simulink model "cable_driven_parallel_robot2022"  (R2022b)
settings: Solver=ode3  StartTime=0.0  StopTime=100  FixedStep=0.01  RelTol=1e-3
values from neighbouring files (symbols this model uses):
  cable_length = 1.2    [Model_Info.m]
  g = 9.81    [Model_Info.m]
  MP_H = 2    [Model_Info.m]
  MP_init_X = 0    [Model_Info.m]
  MP_init_Y = 0    [Model_Info.m]
  MP_init_Z = cable_length + (MP_H/2)    (= 2.2)    [Model_Info.m]
  MP_Ix = (MP_m/12)*(MP_W^2+MP_H^2)    (= 6.66666666667e-05)    [Model_Info.m]
  MP_Iy = (MP_m/12)*(MP_L^2+MP_H^2)    (= 6.66666666667e-05)    [Model_Info.m]
  MP_Iz = (MP_m/12)*(MP_L^2+MP_W^2)    (= 6.66666666667e-05)    [Model_Info.m]
  MP_L = 2    [Model_Info.m]
  MP_m = 0.0001    [Model_Info.m]
  MP_W = 2    [Model_Info.m]
  MR_init_X_L1 = -(MP_L/2)    (= -1)    [Model_Info.m]
  MR_init_X_L2 = (MP_L/2)    (= 1)    [Model_Info.m]
  MR_init_X_L3 = (MP_L/2)    (= 1)    [Model_Info.m]
  MR_init_X_L4 = -(MP_L/2)    (= -1)    [Model_Info.m]
  MR_init_Y_L1 = -(MP_W/2)    (= -1)    [Model_Info.m]
  MR_init_Y_L2 = -(MP_W/2)    (= -1)    [Model_Info.m]
  MR_init_Y_L3 = (MP_W/2)    (= 1)    [Model_Info.m]
  MR_init_Y_L4 = (MP_W/2)    (= 1)    [Model_Info.m]
  MR_init_Yaw_L1 = pi    (= 3.14159265359)    [Model_Info.m]
  MR_init_Yaw_L2 = 0    [Model_Info.m]
  MR_init_Yaw_L3 = 0    [Model_Info.m]
  MR_init_Yaw_L4 = pi    (= 3.14159265359)    [Model_Info.m]
  MR_Jr = (MR_m/12)*(MR_L^2+MR_W^2)    (= 0.333333333333)    [Model_Info.m]
  MR_m = 0.5    [Model_Info.m]
  MR_r = 2    [Model_Info.m]
  MR_WT = 2    [Model_Info.m]
  QR_Ax = 0.25*0    (= 0)    [Model_Info.m]
  QR_Ay = 0.25*0    (= 0)    [Model_Info.m]
  QR_Az = 0.25*0    (= 0)    [Model_Info.m]
  QR_b = 1.14*1e-7    (= 1.14e-07)    [Model_Info.m]
  QR_Ixx = 4.856*1e-3    (= 0.004856)    [Model_Info.m]
  QR_Iyy = 4.856*1e-3    (= 0.004856)    [Model_Info.m]
  QR_Izz = 8.801*1e-3    (= 0.008801)    [Model_Info.m]
  QR_K = 2.980*1e-6    (= 2.98e-06)    [Model_Info.m]
  QR_l = 0.225    [Model_Info.m]
  QR_m = 0.468    [Model_Info.m]
  QR_x0_U1 = -(MP_L/2)    (= -1)    [Model_Info.m]
  QR_x0_U2 = (MP_L/2)    (= 1)    [Model_Info.m]
  QR_x0_U3 = (MP_L/2)    (= 1)    [Model_Info.m]
  QR_x0_U4 = -(MP_L/2)    (= -1)    [Model_Info.m]
  QR_y0_U1 = -(MP_W/2)    (= -1)    [Model_Info.m]
  QR_y0_U2 = -(MP_W/2)    (= -1)    [Model_Info.m]
  QR_y0_U3 = (MP_W/2)    (= 1)    [Model_Info.m]
  QR_y0_U4 = (MP_W/2)    (= 1)    [Model_Info.m]
  QR_z0_U1 = 2*cable_length+(MP_H)    (= 4.4)    [Model_Info.m]
  QR_z0_U2 = 2*cable_length+(MP_H)    (= 4.4)    [Model_Info.m]
  QR_z0_U3 = 2*cable_length+(MP_H)    (= 4.4)    [Model_Info.m]
  QR_z0_U4 = 2*cable_length+(MP_H)    (= 4.4)    [Model_Info.m]
(part 8 of 12)

== matlab function cable_driven_parallel_robot2022/Actuators-CableTension-MovingPlatform/QuadRotor3/Subsystem/QuadCopter Model ==
  data: vx input; x_ddot output size=1; vy input; vz input; phidot input; thetadot input; psidot input; y_ddot output size=1; z_ddot output size=1; phi_ddot output size=1; theta_ddot output size=1; psi_ddot output size=1; phi input; theta input; psi input; constants input; z input; rest output
function [x_ddot,y_ddot,z_ddot,phi_ddot,theta_ddot,psi_ddot,rest] = fcn(vx,vy,vz,phidot,thetadot,psidot, phi,theta,psi,constants,z)
rest=0;
m = constants(1);
g = constants(2);
Ixx = constants(3);
Iyy = constants(4);
Izz = constants(5);
l = constants(6);
K = constants(7);
b = constants(8);
Ax = constants(9);
Ay = constants(10);
Az = constants(11);
omega1 = constants(12);
omega2 = constants(13);
omega3 = constants(14);
omega4 = constants(15);
Tx = constants(16);
Ty = constants(17);
Tz = constants(18);
% x_ddot = (K*omega1^2*sin(phi)*sin(psi) - Ax*vx + K*omega2^2*sin(phi)*sin(psi) + K*omega3^2*sin(phi)*sin(psi) + K*omega4^2*sin(phi)*sin(psi) + K*omega1^2*cos(phi)*cos(psi)*sin(theta) + K*omega2^2*cos(phi)*cos(psi)*sin(theta) + K*omega3^2*cos(phi)*cos(psi)*sin(theta) + K*omega4^2*cos(phi)*cos(psi)*sin(theta))/m;
% y_ddot = -(Ay*vy + K*omega1^2*cos(psi)*sin(phi) + K*omega2^2*cos(psi)*sin(phi) + K*omega3^2*cos(psi)*sin(phi) + K*omega4^2*cos(psi)*sin(phi) - K*omega1^2*cos(phi)*sin(psi)*sin(theta) - K*omega2^2*cos(phi)*sin(psi)*sin(theta) - K*omega3^2*cos(phi)*sin(psi)*sin(theta) - K*omega4^2*cos(phi)*sin(psi)*sin(theta))/m;
% z_ddot = (K*cos(phi)*cos(theta)*omega1^2 + K*cos(phi)*cos(theta)*omega2^2 + K*cos(phi)*cos(theta)*omega3^2 + K*cos(phi)*cos(theta)*omega4^2 - Az*vz - g*m)/m;
% phi_ddot = (2*Ixx*Iyy*b*omega1^2*sin(theta) - 2*Ixx*Iyy*b*omega2^2*sin(theta) + 2*Ixx*Iyy*b*omega3^2*sin(theta) - 2*Ixx*Iyy*b*omega4^2*sin(theta) + 2*Iyy^3*psidot^2*cos(phi)*cos(theta)^4*sin(phi)^3 - 2*Iyy^3*psidot^2*cos(phi)*cos(theta)^4*sin(phi)^5 - 2*Iyy^3*psidot*thetadot*cos(theta)^3*sin(phi)^2 + 2*Iyy^3*psidot*thetadot*cos(theta)^3*sin(phi)^4 - 2*Iyy^3*psidot^2*cos(phi)^3*cos(theta)^4*sin(phi)^3 - Iyy^3*thetadot^2*sin(2*phi)*cos(theta)^2*sin(phi)^2 + Iyy^3*thetadot^2*sin(2*phi)*cos(theta)^2*sin(phi)^4 - Ixx*Iyy^2*thetadot^2*sin(2*phi)*sin(theta)^2 - 2*Iyy^2*K*l*omega2^2*cos(theta)^2*sin(phi)^2 + 2*Iyy^2*K*l*omega2^2*cos(theta)^2*sin(phi)^4 + 2*Iyy^2*K*l*omega4^2*cos(theta)^2*sin(phi)^2 - 2*Iyy^2*K*l*omega4^2*cos(theta)^2*sin(phi)^4 + 2*Ixx*Iyy^2*thetadot^2*cos(phi)*sin(phi)*sin(theta)^2 - 2*Ixx*Iyy*b*omega1^2*sin(phi)^2*sin(theta) + 2*Ixx*Iyy*b*omega2^2*sin(phi)^2*sin(theta) - 2*Ixx*Iyy*b*omega3^2*sin(phi)^2*sin(theta) + 2*Ixx*Iyy*b*omega4^2*sin(phi)^2*sin(theta) + 2*Ixx*Izz*b*omega1^2*sin(phi)^2*sin(theta) - 2*Ixx*Izz*b*omega2^2*sin(phi)^2*sin(theta) + 2*Ixx*Izz*b*omega3^2*sin(phi)^2*sin(theta) - 2*Ixx*Izz*b*omega4^2*sin(phi)^2*sin(theta) - 2*Ixx*Iyy^2*psidot*thetadot*cos(theta)*sin(theta)^2 + 2*Ixx^2*Iyy*psidot*thetadot*cos(theta)*sin(theta)^2 + 2*Ixx*Iyy^2*psidot*thetadot*sin(2*theta)*sin(theta) - 2*Ixx^2*Iyy*psidot*thetadot*sin(2*theta)*sin(theta) - 2*Iyy*Izz^2*psidot^2*cos(phi)^3*cos(theta)^4*sin(phi) - 2*Iyy^2*Izz*psidot^2*cos(phi)*cos(theta)^4*sin(phi)^3 + 2*Iyy^2*Izz*psidot^2*cos(phi)^3*cos(theta)^4*sin(phi) - 2*Iyy*Izz^2*psidot^2*cos(phi)*cos(theta)^4*sin(phi)^5 + 4*Iyy^2*Izz*psidot^2*cos(phi)*cos(theta)^4*sin(phi)^5 - 2*Ixx*Iyy^2*thetadot^2*cos(phi)*sin(phi)^3*sin(theta)^2 - 2*Ixx*Izz^2*thetadot^2*cos(phi)*sin(phi)^3*sin(theta)^2 + Ixx*Iyy*Izz*thetadot^2*sin(2*phi)*sin(theta)^2 + 6*Iyy^3*psidot*thetadot*cos(phi)^2*cos(theta)^3*sin(phi)^2 - 4*Iyy^3*psidot*thetadot*cos(phi)^2*cos(theta)^3*sin(phi)^4 - 4*Iyy^3*psidot*thetadot*cos(phi)^4*cos(theta)^3*sin(phi)^2 + 2*Iyy*Izz^2*psidot*thetadot*cos(phi)^2*cos(theta)^3 - 2*Iyy^2*Izz*psidot*thetadot*cos(phi)^2*cos(theta)^3 - 4*Iyy*Izz^2*psidot*thetadot*cos(phi)^4*cos(theta)^3 + 4*Iyy^2*Izz*psidot*thetadot*cos(phi)^4*cos(theta)^3 + 2*Ixx*Iyy^2*psidot*thetadot*cos(theta)^3*sin(phi)^2 - 2*Ixx*Iyy^2*psidot*thetadot*cos(theta)^3*sin(phi)^4 + 2*Iyy^2*Izz*psidot*thetadot*cos(theta)^3*sin(phi)^2 + 2*Iyy*Izz^2*psidot*thetadot*cos(theta)^3*sin(phi)^4 - 4*Iyy^2*Izz*psidot*thetadot*cos(theta)^3*sin(phi)^4 - 2*Ixx*Iyy*K*l*omega2^2*sin(theta)^2 + 2*Ixx*Iyy*K*l*omega4^2*sin(theta)^2 + Iyy^3*thetadot^2*sin(2*phi)*cos(phi)^2*cos(theta)^2*sin(phi)^2 - 2*Iyy*Izz^2*psidot^2*cos(phi)^3*cos(theta)^4*sin(phi)^3 + 4*Iyy^2*Izz*psidot^2*cos(phi)^3*cos(theta)^4*sin(phi)^3 + Iyy*Izz^2*thetadot^2*sin(2*phi)*cos(phi)^2*cos(theta)^2 - Iyy^2*Izz*thetadot^2*sin(2*phi)*cos(phi)^2*cos(theta)^2 + Iyy^2*Izz*thetadot^2*sin(2*phi)*cos(theta)^2*sin(phi)^2 + Iyy*Izz^2*thetadot^2*sin(2*phi)*cos(theta)^2*sin(phi)^4 - 2*Iyy^2*Izz*thetadot^2*sin(2*phi)*cos(theta)^2*sin(phi)^4 + Ixx*Iyy^2*thetadot^2*sin(2*phi)*sin(phi)^2*sin(theta)^2 + Ixx*Izz^2*thetadot^2*sin(2*phi)*sin(phi)^2*sin(theta)^2 + 2*Ixx*Iyy^2*phidot*thetadot*cos(theta)*sin(theta) + 2*Ixx^2*Iyy*phidot*thetadot*cos(theta)*sin(theta) + 2*Ixx*Iyy*K*l*omega2^2*sin(phi)^2*sin(theta)^2 - 2*Ixx*Iyy*K*l*omega4^2*sin(phi)^2*sin(theta)^2 - 2*Ixx*Izz*K*l*omega2^2*sin(phi)^2*sin(theta)^2 + 2*Ixx*Izz*K*l*omega4^2*sin(phi)^2*sin(theta)^2 - 2*Ixx*Iyy*Izz*thetadot^2*cos(phi)*sin(phi)*sin(theta)^2 + Iyy*Izz^2*thetadot^2*sin(2*phi)*cos(phi)^2*cos(theta)^2*sin(phi)^2 - 2*Iyy^2*Izz*thetadot^2*sin(2*phi)*cos(phi)^2*cos(theta)^2*sin(phi)^2 - 4*Ixx*Iyy^2*phidot*thetadot*cos(phi)^2*cos(theta)*sin(theta) - 2*Ixx*Iyy^2*phidot*thetadot*cos(theta)*sin(phi)^2*sin(theta) - 2*Ixx^2*Iyy*phidot*thetadot*cos(theta)*sin(phi)^2*sin(theta) - 2*Ixx*Izz^2*phidot*thetadot*cos(theta)*sin(phi)^2*sin(theta) + 2*Ixx^2*Izz*phidot*thetadot*cos(theta)*sin(phi)^2*sin(theta) + 2*Iyy^2*K*l*omega2^2*cos(phi)^2*cos(theta)^2*sin(phi)^2 - 2*Iyy^2*K*l*omega4^2*cos(phi)^2*cos(theta)^2*sin(phi)^2 + 2*Ixx*Iyy*Izz*psidot*thetadot*cos(theta)*sin(theta)^2 + 2*Ixx*Iyy^2*psidot^2*cos(phi)*cos(theta)^2*sin(phi)*sin(theta)^2 + 4*Ixx*Iyy*Izz*thetadot^2*cos(phi)*sin(phi)^3*sin(theta)^2 + 2*Ixx*Iyy*Izz*psidot*thetadot*cos(phi)^2*cos(theta)^3 + 2*Ixx*Iyy^2*psidot*thetadot*cos(theta)*sin(phi)^2*sin(theta)^2 - 2*Ixx^2*Iyy*psidot*thetadot*cos(theta)*sin(phi)^2*sin(theta)^2 + 2*Ixx*Izz^2*psidot*thetadot*cos(theta)*sin(phi)^2*sin(theta)^2 + 2*Ixx^2*Izz*psidot*thetadot*cos(theta)*sin(phi)^2*sin(theta)^2 + 2*Ixx*Iyy*Izz*psidot*thetadot*cos(theta)^3*sin(phi)^4 - 2*Ixx*Iyy^2*psidot*thetadot*sin(2*theta)*sin(phi)^2*sin(theta) + 2*Ixx^2*Iyy*psidot*thetadot*sin(2*theta)*sin(phi)^2*sin(theta) - 2*Ixx^2*Izz*psidot*thetadot*sin(2*theta)*sin(phi)^2*sin(theta) - 2*Ixx*Izz^2*psidot^2*cos(phi)*cos(theta)^2*sin(phi)^3*sin(theta)^2 - 2*Ixx*Izz^2*psidot^2*cos(phi)^3*cos(theta)^2*sin(phi)*sin(theta)^2 - 2*Ixx*Iyy*Izz*thetadot^2*sin(2*phi)*sin(phi)^2*sin(theta)^2 - 2*Ixx*Iyy*Izz*phidot*thetadot*cos(theta)*sin(theta) - 2*Iyy*Izz*K*l*omega2^2*cos(phi)^2*cos(theta)^2 + 2*Iyy*Izz*K*l*omega4^2*cos(phi)^2*cos(theta)^2 - 2*Ixx*Iyy^2*psidot*thetadot*cos(phi)^2*cos(theta)^3*sin(phi)^2 + 2*Iyy*Izz^2*psidot*thetadot*cos(phi)^2*cos(theta)^3*sin(phi)^2 - 8*Iyy^2*Izz*psidot*thetadot*cos(phi)^2*cos(theta)^3*sin(phi)^2 - 4*Iyy*Izz^2*psidot*thetadot*cos(phi)^2*cos(theta)^3*sin(phi)^4 - 4*Iyy*Izz^2*psidot*thetadot*cos(phi)^4*cos(theta)^3*sin(phi)^2 + 8*Iyy^2*Izz*psidot*thetadot*cos(phi)^2*cos(theta)^3*sin(phi)^4 + 8*Iyy^2*Izz*psidot*thetadot*cos(phi)^4*cos(theta)^3*sin(phi)^2 - 2*Iyy*Izz*K*l*omega2^2*cos(theta)^2*sin(phi)^4 + 2*Iyy*Izz*K*l*omega4^2*cos(theta)^2*sin(phi)^4 - 4*Ixx*Iyy^2*phidot*psidot*cos(phi)*cos(theta)^2*sin(phi)*sin(theta) + 2*Ixx^2*Iyy*phidot*psidot*cos(phi)*cos(theta)^2*sin(phi)*sin(theta) - 2*Ixx^2*Izz*phidot*psidot*cos(phi)*cos(theta)^2*sin(phi)*sin(theta) + 4*Ixx*Iyy*Izz*phidot*thetadot*cos(phi)^2*cos(theta)*sin(theta) + 4*Ixx*Iyy*Izz*phidot*thetadot*cos(theta)*sin(phi)^2*sin(theta) - 2*Iyy*Izz*K*l*omega2^2*cos(phi)^2*cos(theta)^2*sin(phi)^2 + 2*Iyy*Izz*K*l*omega4^2*cos(phi)^2*cos(theta)^2*sin(phi)^2 - 2*Ixx*Iyy*Izz*psidot^2*cos(phi)*cos(theta)^2*sin(phi)*sin(theta)^2 + 2*Ixx*Iyy^2*phidot*psidot*cos(phi)*cos(theta)^2*sin(phi)^3*sin(theta) + 2*Ixx*Iyy^2*phidot*psidot*cos(phi)^3*cos(theta)^2*sin(phi)*sin(theta) + 2*Ixx*Izz^2*phidot*psidot*cos(phi)*cos(theta)^2*sin(phi)^3*sin(theta) + 2*Ixx*Izz^2*phidot*psidot*cos(phi)^3*cos(theta)^2*sin(phi)*sin(theta) + 4*Ixx*Iyy^2*phidot*thetadot*cos(phi)^2*cos(theta)*sin(phi)^2*sin(theta) + 4*Ixx*Izz^2*phidot*thetadot*cos(phi)^2*cos(theta)*sin(phi)^2*sin(theta) - 4*Ixx*Iyy*Izz*psidot*thetadot*cos(theta)*sin(phi)^2*sin(theta)^2 + 2*Ixx*Iyy*Izz*psidot*thetadot*sin(2*theta)*sin(phi)^2*sin(theta) + 2*Ixx*Iyy*Izz*psidot^2*cos(phi)*cos(theta)^2*sin(phi)^3*sin(theta)^2 + 2*Ixx*Iyy*Izz*psidot^2*cos(phi)^3*cos(theta)^2*sin(phi)*sin(theta)^2 + 2*Ixx*Iyy*Izz*psidot*thetadot*cos(phi)^2*cos(theta)^3*sin(phi)^2 - Ixx^2*Iyy*psidot^2*sin(2*theta)*cos(phi)*cos(theta)*sin(phi)*sin(theta) + Ixx^2*Izz*psidot^2*sin(2*theta)*cos(phi)*cos(theta)*sin(phi)*sin(theta) - 4*Ixx*Iyy*Izz*phidot*psidot*cos(phi)*cos(theta)^2*sin(phi)^3*sin(theta) - 4*Ixx*Iyy*Izz*phidot*psidot*cos(phi)^3*cos(theta)^2*sin(phi)*sin(theta) - 8*Ixx*Iyy*Izz*phidot*thetadot*cos(phi)^2*cos(theta)*sin(phi)^2*sin(theta) + 2*Ixx*Iyy*K*l*omega1^2*cos(phi)*cos(theta)*sin(phi)*sin(theta) - 2*Ixx*Iyy*K*l*omega3^2*cos(phi)*cos(theta)*sin(phi)*sin(theta) - 2*Ixx*Izz*K*l*omega1^2*cos(phi)*cos(theta)*sin(phi)*sin(theta) + 2*Ixx*Izz*K*l*omega3^2*cos(phi)*cos(theta)*sin(phi)*sin(theta) - 2*Ixx*Iyy^2*phidot*thetadot*sin(2*phi)*cos(phi)*cos(theta)*sin(phi)*sin(theta) - 2*Ixx*Izz^2*phidot*thetadot*sin(2*phi)*cos(phi)*cos(theta)*sin(phi)*sin(theta) + 4*Ixx*Iyy*Izz*phidot*psidot*cos(phi)*cos(theta)^2*sin(phi)*sin(theta) + 4*Ixx*Iyy*Izz*phidot*thetadot*sin(2*phi)*cos(phi)*cos(theta)*sin(phi)*sin(theta))/(2*Ixx*cos(theta)^2*(- Iyy^2*cos(phi)^2*sin(phi)^2 - Iyy^2*sin(phi)^4 + Iyy^2*sin(phi)^2 + Izz*Iyy*cos(phi)^2*sin(phi)^2 + Izz*Iyy*cos(phi)^2 + Izz*Iyy*sin(phi)^4));
% theta_ddot = -(2*Izz^2*psidot^2*cos(phi)^4*cos(theta)^2*sin(theta) + 2*Iyy^2*thetadot^2*cos(phi)^2*sin(phi)^2*sin(theta) + 2*Izz^2*thetadot^2*cos(phi)^2*sin(phi)^2*sin(theta) + 2*Iyy^2*psidot^2*cos(theta)^2*sin(phi)^4*sin(theta) - 2*Izz^2*phidot*psidot*cos(phi)^4*cos(theta)^2 - 2*Iyy^2*phidot*psidot*cos(theta)^2*sin(phi)^4 + 2*Iyy*b*omega1^2*cos(phi)*sin(phi) - 2*Iyy*b*omega2^2*cos(phi)*sin(phi) + 2*Iyy*b*omega3^2*cos(phi)*sin(phi) - 2*Iyy*b*omega4^2*cos(phi)*sin(phi) - 2*Izz*b*omega1^2*cos(phi)*sin(phi) + 2*Izz*b*omega2^2*cos(phi)*sin(phi) - 2*Izz*b*omega3^2*cos(phi)*sin(phi) + 2*Izz*b*omega4^2*cos(phi)*sin(phi) - Ixx*Izz*psidot^2*sin(2*theta)*cos(phi)^2*cos(theta) - 4*Iyy*Izz*thetadot^2*cos(phi)^2*sin(phi)^2*sin(theta) - Ixx*Iyy*psidot^2*sin(2*theta)*cos(theta)*sin(phi)^2 + 2*Izz*K*l*omega1^2*cos(phi)^2*cos(theta) - 2*Izz*K*l*omega3^2*cos(phi)^2*cos(theta) + 2*Izz^2*phidot*thetadot*sin(2*phi)*cos(phi)^2*cos(theta) + 2*Ixx*Izz*phidot*psidot*cos(phi)^2*cos(theta)^2 + 2*Iyy*Izz*phidot*psidot*cos(phi)^4*cos(theta)^2 + 2*Iyy*K*l*omega1^2*cos(theta)*sin(phi)^2 - 2*Iyy*K*l*omega3^2*cos(theta)*sin(phi)^2 - 2*Iyy^2*phidot*thetadot*sin(2*phi)*cos(theta)*sin(phi)^2 + 2*Ixx*Iyy*phidot*psidot*cos(theta)^2*sin(phi)^2 + 2*Iyy*Izz*phidot*psidot*cos(theta)^2*sin(phi)^4 + 2*Iyy^2*psidot^2*cos(phi)^2*cos(theta)^2*sin(phi)^2*sin(theta) + 2*Izz^2*psidot^2*cos(phi)^2*cos(theta)^2*sin(phi)^2*sin(theta) + 2*Iyy^2*phidot*thetadot*cos(phi)*cos(theta)*sin(phi) + 2*Izz^2*phidot*thetadot*cos(phi)*cos(theta)*sin(phi) - 2*Iyy^2*phidot*psidot*cos(phi)^2*cos(theta)^2*sin(phi)^2 - 2*Izz^2*phidot*psidot*cos(phi)^2*cos(theta)^2*sin(phi)^2 - Iyy^2*thetadot^2*sin(2*phi)*cos(phi)*sin(phi)*sin(theta) - Izz^2*thetadot^2*sin(2*phi)*cos(phi)*sin(phi)*sin(theta) - 4*Iyy^2*phidot*thetadot*cos(phi)^3*cos(theta)*sin(phi) - 4*Izz^2*phidot*thetadot*cos(phi)^3*cos(theta)*sin(phi) + 2*Iyy^2*psidot*thetadot*sin(2*theta)*cos(phi)*sin(phi) - 2*Iyy*Izz*phidot*thetadot*sin(2*phi)*cos(phi)^2*cos(theta) + 2*Iyy*Izz*phidot*thetadot*sin(2*phi)*cos(theta)*sin(phi)^2 - 2*Iyy^2*psidot*thetadot*cos(phi)*cos(theta)*sin(phi)*sin(theta) - 2*Izz^2*psidot*thetadot*cos(phi)*cos(theta)*sin(phi)*sin(theta) + 2*Ixx*Iyy*phidot*thetadot*cos(phi)*cos(theta)*sin(phi) - 2*Ixx*Izz*phidot*thetadot*cos(phi)*cos(theta)*sin(phi) - 4*Iyy*Izz*phidot*thetadot*cos(phi)*cos(theta)*sin(phi) + 4*Iyy*Izz*phidot*psidot*cos(phi)^2*cos(theta)^2*sin(phi)^2 + 2*Iyy*Izz*thetadot^2*sin(2*phi)*cos(phi)*sin(phi)*sin(theta) + 8*Iyy*Izz*phidot*thetadot*cos(phi)^3*cos(theta)*sin(phi) - 2*Iyy*K*l*omega2^2*cos(phi)*sin(phi)*sin(theta) + 2*Iyy*K*l*omega4^2*cos(phi)*sin(phi)*sin(theta) + 2*Izz*K*l*omega2^2*cos(phi)*sin(phi)*sin(theta) - 2*Izz*K*l*omega4^2*cos(phi)*sin(phi)*sin(theta) - 2*Ixx*Iyy*psidot*thetadot*sin(2*theta)*cos(phi)*sin(phi) + 2*Ixx*Izz*psidot*thetadot*sin(2*theta)*cos(phi)*sin(phi) - 2*Iyy*Izz*psidot*thetadot*sin(2*theta)*cos(phi)*sin(phi) + 2*Ixx*Iyy*psidot*thetadot*cos(phi)*cos(theta)*sin(phi)*sin(theta) - 2*Ixx*Izz*psidot*thetadot*cos(phi)*cos(theta)*sin(phi)*sin(theta) + 4*Iyy*Izz*psidot*thetadot*cos(phi)*cos(theta)*sin(phi)*sin(theta))/(2*cos(theta)*(- Iyy^2*cos(phi)^2*sin(phi)^2 - Iyy^2*sin(phi)^4 + Iyy^2*sin(phi)^2 + Izz*Iyy*cos(phi)^2*sin(phi)^2 + Izz*Iyy*cos(phi)^2 + Izz*Iyy*sin(phi)^4));
% psi_ddot = (2*Iyy*b*omega1^2 - 2*Iyy*b*omega2^2 + 2*Iyy*b*omega3^2 - 2*Iyy*b*omega4^2 - Iyy^2*thetadot^2*sin(2*phi)*sin(theta) - 2*Iyy*b*omega1^2*sin(phi)^2 + 2*Iyy*b*omega2^2*sin(phi)^2 - 2*Iyy*b*omega3^2*sin(phi)^2 + 2*Iyy*b*omega4^2*sin(phi)^2 + 2*Izz*b*omega1^2*sin(phi)^2 - 2*Izz*b*omega2^2*sin(phi)^2 + 2*Izz*b*omega3^2*sin(phi)^2 - 2*Izz*b*omega4^2*sin(phi)^2 + 2*Iyy^2*psidot*thetadot*sin(2*theta) + 2*Iyy^2*phidot*thetadot*cos(theta) - 2*Iyy^2*phidot*thetadot*cos(theta)*sin(phi)^2 - 2*Izz^2*phidot*thetadot*cos(theta)*sin(phi)^2 - 2*Iyy*K*l*omega2^2*sin(theta) + 2*Iyy*K*l*omega4^2*sin(theta) - 2*Ixx*Iyy*psidot*thetadot*sin(2*theta) + Iyy^2*thetadot^2*sin(2*phi)*sin(phi)^2*sin(theta) + Izz^2*thetadot^2*sin(2*phi)*sin(phi)^2*sin(theta) - 2*Iyy^2*psidot*thetadot*sin(2*theta)*sin(phi)^2 + 2*Iyy^2*thetadot^2*cos(phi)*sin(phi)*sin(theta) - 2*Iyy^2*psidot*thetadot*cos(theta)*sin(theta) + 2*Ixx*Iyy*phidot*thetadot*cos(theta) - 2*Iyy*Izz*phidot*thetadot*cos(theta) - 2*Iyy^2*thetadot^2*cos(phi)*sin(phi)^3*sin(theta) - 2*Izz^2*thetadot^2*cos(phi)*sin(phi)^3*sin(theta) + Iyy*Izz*thetadot^2*sin(2*phi)*sin(theta) - 4*Iyy^2*phidot*thetadot*cos(phi)^2*cos(theta) - 2*Izz^2*psidot^2*cos(phi)*cos(theta)^2*sin(phi)^3*sin(theta) - 2*Izz^2*psidot^2*cos(phi)^3*cos(theta)^2*sin(phi)*sin(theta) - 2*Iyy*Izz*thetadot^2*sin(2*phi)*sin(phi)^2*sin(theta) + 2*Iyy^2*phidot*psidot*cos(phi)*cos(theta)^2*sin(phi)^3 + 2*Iyy^2*phidot*psidot*cos(phi)^3*cos(theta)^2*sin(phi) + 2*Izz^2*phidot*psidot*cos(phi)*cos(theta)^2*sin(phi)^3 + 2*Izz^2*phidot*psidot*cos(phi)^3*cos(theta)^2*sin(phi) + 4*Iyy^2*phidot*thetadot*cos(phi)^2*cos(theta)*sin(phi)^2 + 4*Izz^2*phidot*thetadot*cos(phi)^2*cos(theta)*sin(phi)^2 + 2*Iyy*K*l*omega2^2*sin(phi)^2*sin(theta) - 2*Iyy*K*l*omega4^2*sin(phi)^2*sin(theta) - 2*Izz*K*l*omega2^2*sin(phi)^2*sin(theta) + 2*Izz*K*l*omega4^2*sin(phi)^2*sin(theta) + 2*Ixx*Iyy*psidot*thetadot*sin(2*theta)*sin(phi)^2 - 2*Ixx*Izz*psidot*thetadot*sin(2*theta)*sin(phi)^2 + 2*Iyy*Izz*psidot*thetadot*sin(2*theta)*sin(phi)^2 - 2*Iyy*Izz*thetadot^2*cos(phi)*sin(phi)*sin(theta) + 2*Ixx*Iyy*psidot*thetadot*cos(theta)*sin(theta) + 2*Iyy*Izz*psidot*thetadot*cos(theta)*sin(theta) + 2*Iyy^2*psidot^2*cos(phi)*cos(theta)^2*sin(phi)*sin(theta) + 4*Iyy*Izz*thetadot^2*cos(phi)*sin(phi)^3*sin(theta) - 4*Iyy^2*phidot*psidot*cos(phi)*cos(theta)^2*sin(phi) + 4*Iyy*Izz*phidot*thetadot*cos(phi)^2*cos(theta) + 2*Iyy^2*psidot*thetadot*cos(theta)*sin(phi)^2*sin(theta) + 2*Izz^2*psidot*thetadot*cos(theta)*sin(phi)^2*sin(theta) - 2*Ixx*Iyy*phidot*thetadot*cos(theta)*sin(phi)^2 + 2*Ixx*Izz*phidot*thetadot*cos(theta)*sin(phi)^2 + 4*Iyy*Izz*phidot*thetadot*cos(theta)*sin(phi)^2 - 4*Iyy*Izz*phidot*psidot*cos(phi)*cos(theta)^2*sin(phi)^3 - 4*Iyy*Izz*phidot*psidot*cos(phi)^3*cos(theta)^2*sin(phi) - 8*Iyy*Izz*phidot*thetadot*cos(phi)^2*cos(theta)*sin(phi)^2 - Ixx*Iyy*psidot^2*sin(2*theta)*cos(phi)*cos(theta)*sin(phi) + Ixx*Izz*psidot^2*sin(2*theta)*cos(phi)*cos(theta)*sin(phi) - 2*Iyy*Izz*psidot^2*cos(phi)*cos(theta)^2*sin(phi)*sin(theta) + 2*Iyy*K*l*omega1^2*cos(phi)*cos(theta)*sin(phi) - 2*Iyy*K*l*omega3^2*cos(phi)*cos(theta)*sin(phi) - 2*Izz*K*l*omega1^2*cos(phi)*cos(theta)*sin(phi) + 2*Izz*K*l*omega3^2*cos(phi)*cos(theta)*sin(phi) - 2*Iyy^2*phidot*thetadot*sin(2*phi)*cos(phi)*cos(theta)*sin(phi) - 2*Izz^2*phidot*thetadot*sin(2*phi)*cos(phi)*cos(theta)*sin(phi) + 2*Ixx*Iyy*phidot*psidot*cos(phi)*cos(theta)^2*sin(phi) - 2*Ixx*Izz*phidot*psidot*cos(phi)*cos(theta)^2*sin(phi) + 4*Iyy*Izz*phidot*psidot*cos(phi)*cos(theta)^2*sin(phi) - 2*Ixx*Iyy*psidot*thetadot*cos(theta)*sin(phi)^2*sin(theta) + 2*Ixx*Izz*psidot*thetadot*cos(theta)*sin(phi)^2*sin(theta) - 4*Iyy*Izz*psidot*thetadot*cos(theta)*sin(phi)^2*sin(theta) + 2*Iyy*Izz*psidot^2*cos(phi)*cos(theta)^2*sin(phi)^3*sin(theta) + 2*Iyy*Izz*psidot^2*cos(phi)^3*cos(theta)^2*sin(phi)*sin(theta) + 4*Iyy*Izz*phidot*thetadot*sin(2*phi)*cos(phi)*cos(theta)*sin(phi))/(2*cos(theta)^2*(- Iyy^2*cos(phi)^2*sin(phi)^2 - Iyy^2*sin(phi)^4 + Iyy^2*sin(phi)^2 + Izz*Iyy*cos(phi)^2*sin(phi)^2 + Izz*Iyy*cos(phi)^2 + Izz*Iyy*sin(phi)^4));
x_ddot =  (K*omega1^2*sin(phi)*sin(psi) - Ax*vx + Tx + K*omega2^2*sin(phi)*sin(psi) + K*omega3^2*sin(phi)*sin(psi) + K*omega4^2*sin(phi)*sin(psi) + K*omega1^2*cos(phi)*cos(psi)*sin(theta) + K*omega2^2*cos(phi)*cos(psi)*sin(theta) + K*omega3^2*cos(phi)*cos(psi)*sin(theta) + K*omega4^2*cos(phi)*cos(psi)*sin(theta))/m;
y_ddot = -(-Ty + Ay*vy + K*omega1^2*cos(psi)*sin(phi) + K*omega2^2*cos(psi)*sin(phi) + K*omega3^2*cos(psi)*sin(phi) + K*omega4^2*cos(psi)*sin(phi) - K*omega1^2*cos(phi)*sin(psi)*sin(theta) - K*omega2^2*cos(phi)*sin(psi)*sin(theta) - K*omega3^2*cos(phi)*sin(psi)*sin(theta) - K*omega4^2*cos(phi)*sin(psi)*sin(theta))/m;
z_ddot = (K*cos(phi)*cos(theta)*omega1^2 + K*cos(phi)*cos(theta)*omega2^2 + K*cos(phi)*cos(theta)*omega3^2 + K*cos(phi)*cos(theta)*omega4^2 + Tz - Az*vz - g*m)/m;
phi_ddot = (2*Ixx*Iyy*b*omega1^2*sin(theta) - 2*Ixx*Iyy*b*omega2^2*sin(theta) + 2*Ixx*Iyy*b*omega3^2*sin(theta) - 2*Ixx*Iyy*b*omega4^2*sin(theta) + 2*Iyy^3*psidot^2*cos(phi)*cos(theta)^4*sin(phi)^3 - 2*Iyy^3*psidot^2*cos(phi)*cos(theta)^4*sin(phi)^5 - 2*Iyy^3*psidot*thetadot*cos(theta)^3*sin(phi)^2 + 2*Iyy^3*psidot*thetadot*cos(theta)^3*sin(phi)^4 - 2*Iyy^3*psidot^2*cos(phi)^3*cos(theta)^4*sin(phi)^3 - Iyy^3*thetadot^2*sin(2*phi)*cos(theta)^2*sin(phi)^2 + Iyy^3*thetadot^2*sin(2*phi)*cos(theta)^2*sin(phi)^4 - Ixx*Iyy^2*thetadot^2*sin(2*phi)*sin(theta)^2 - 2*Iyy^2*K*l*omega2^2*cos(theta)^2*sin(phi)^2 + 2*Iyy^2*K*l*omega2^2*cos(theta)^2*sin(phi)^4 + 2*Iyy^2*K*l*omega4^2*cos(theta)^2*sin(phi)^2 - 2*Iyy^2*K*l*omega4^2*cos(theta)^2*sin(phi)^4 + 2*Ixx*Iyy^2*thetadot^2*cos(phi)*sin(phi)*sin(theta)^2 - 2*Ixx*Iyy*b*omega1^2*sin(phi)^2*sin(theta) + 2*Ixx*Iyy*b*omega2^2*sin(phi)^2*sin(theta) - 2*Ixx*Iyy*b*omega3^2*sin(phi)^2*sin(theta) + 2*Ixx*Iyy*b*omega4^2*sin(phi)^2*sin(theta) + 2*Ixx*Izz*b*omega1^2*sin(phi)^2*sin(theta) - 2*Ixx*Izz*b*omega2^2*sin(phi)^2*sin(theta) + 2*Ixx*Izz*b*omega3^2*sin(phi)^2*sin(theta) - 2*Ixx*Izz*b*omega4^2*sin(phi)^2*sin(theta) - 2*Ixx*Iyy^2*psidot*thetadot*cos(theta)*sin(theta)^2 + 2*Ixx^2*Iyy*psidot*thetadot*cos(theta)*sin(theta)^2 + 2*Ixx*Iyy^2*psidot*thetadot*sin(2*theta)*sin(theta) - 2*Ixx^2*Iyy*psidot*thetadot*sin(2*theta)*sin(theta) - 2*Iyy*Izz^2*psidot^2*cos(phi)^3*cos(theta)^4*sin(phi) - 2*Iyy^2*Izz*psidot^2*cos(phi)*cos(theta)^4*sin(phi)^3 + 2*Iyy^2*Izz*psidot^2*cos(phi)^3*cos(theta)^4*sin(phi) - 2*Iyy*Izz^2*psidot^2*cos(phi)*cos(theta)^4*sin(phi)^5 + 4*Iyy^2*Izz*psidot^2*cos(phi)*cos(theta)^4*sin(phi)^5 - 2*Ixx*Iyy^2*thetadot^2*cos(phi)*sin(phi)^3*sin(theta)^2 - 2*Ixx*Izz^2*thetadot^2*cos(phi)*sin(phi)^3*sin(theta)^2 + Ixx*Iyy*Izz*thetadot^2*sin(2*phi)*sin(theta)^2 + 6*Iyy^3*psidot*thetadot*cos(phi)^2*cos(theta)^3*sin(phi)^2 - 4*Iyy^3*psidot*thetadot*cos(phi)^2*cos(theta)^3*sin(phi)^4 - 4*Iyy^3*psidot*thetadot*cos(phi)^4*cos(theta)^3*sin(phi)^2 + 2*Iyy*Izz^2*psidot*thetadot*cos(phi)^2*cos(theta)^3 - 2*Iyy^2*Izz*psidot*thetadot*cos(phi)^2*cos(theta)^3 - 4*Iyy*Izz^2*psidot*thetadot*cos(phi)^4*cos(theta)^3 + 4*Iyy^2*Izz*psidot*thetadot*cos(phi)^4*cos(theta)^3 + 2*Ixx*Iyy^2*psidot*thetadot*cos(theta)^3*sin(phi)^2 - 2*Ixx*Iyy^2*psidot*thetadot*cos(theta)^3*sin(phi)^4 + 2*Iyy^2*Izz*psidot*thetadot*cos(theta)^3*sin(phi)^2 + 2*Iyy*Izz^2*psidot*thetadot*cos(theta)^3*sin(phi)^4 - 4*Iyy^2*Izz*psidot*thetadot*cos(theta)^3*sin(phi)^4 - 2*Ixx*Iyy*K*l*omega2^2*sin(theta)^2 + 2*Ixx*Iyy*K*l*omega4^2*sin(theta)^2 + Iyy^3*thetadot^2*sin(2*phi)*cos(phi)^2*cos(theta)^2*sin(phi)^2 - 2*Iyy*Izz^2*psidot^2*cos(phi)^3*cos(theta)^4*sin(phi)^3 + 4*Iyy^2*Izz*psidot^2*cos(phi)^3*cos(theta)^4*sin(phi)^3 + Iyy*Izz^2*thetadot^2*sin(2*phi)*cos(phi)^2*cos(theta)^2 - Iyy^2*Izz*thetadot^2*sin(2*phi)*cos(phi)^2*cos(theta)^2 + Iyy^2*Izz*thetadot^2*sin(2*phi)*cos(theta)^2*sin(phi)^2 + Iyy*Izz^2*thetadot^2*sin(2*phi)*cos(theta)^2*sin(phi)^4 - 2*Iyy^2*Izz*thetadot^2*sin(2*phi)*cos(theta)^2*sin(phi)^4 + Ixx*Iyy^2*thetadot^2*sin(2*phi)*sin(phi)^2*sin(theta)^2 + Ixx*Izz^2*thetadot^2*sin(2*phi)*sin(phi)^2*sin(theta)^2 + 2*Ixx*Iyy^2*phidot*thetadot*cos(theta)*sin(theta) + 2*Ixx^2*Iyy*phidot*thetadot*cos(theta)*sin(theta) + 2*Ixx*Iyy*K*l*omega2^2*sin(phi)^2*sin(theta)^2 - 2*Ixx*Iyy*K*l*omega4^2*sin(phi)^2*sin(theta)^2 - 2*Ixx*Izz*K*l*omega2^2*sin(phi)^2*sin(theta)^2 + 2*Ixx*Izz*K*l*omega4^2*sin(phi)^2*sin(theta)^2 - 2*Ixx*Iyy*Izz*thetadot^2*cos(phi)*sin(phi)*sin(theta)^2 + Iyy*Izz^2*thetadot^2*sin(2*phi)*cos(phi)^2*cos(theta)^2*sin(phi)^2 - 2*Iyy^2*Izz*thetadot^2*sin(2*phi)*cos(phi)^2*cos(theta)^2*sin(phi)^2 - 4*Ixx*Iyy^2*phidot*thetadot*cos(phi)^2*cos(theta)*sin(theta) - 2*Ixx*Iyy^2*phidot*thetadot*cos(theta)*sin(phi)^2*sin(theta) - 2*Ixx^2*Iyy*phidot*thetadot*cos(theta)*sin(phi)^2*sin(theta) - 2*Ixx*Izz^2*phidot*thetadot*cos(theta)*sin(phi)^2*sin(theta) + 2*Ixx^2*Izz*phidot*thetadot*cos(theta)*sin(phi)^2*sin(theta) + 2*Iyy^2*K*l*omega2^2*cos(phi)^2*cos(theta)^2*sin(phi)^2 - 2*Iyy^2*K*l*omega4^2*cos(phi)^2*cos(theta)^2*sin(phi)^2 + 2*Ixx*Iyy*Izz*psidot*thetadot*cos(theta)*sin(theta)^2 + 2*Ixx*Iyy^2*psidot^2*cos(phi)*cos(theta)^2*sin(phi)*sin(theta)^2 + 4*Ixx*Iyy*Izz*thetadot^2*cos(phi)*sin(phi)^3*sin(theta)^2 + 2*Ixx*Iyy*Izz*psidot*thetadot*cos(phi)^2*cos(theta)^3 + 2*Ixx*Iyy^2*psidot*thetadot*cos(theta)*sin(phi)^2*sin(theta)^2 - 2*Ixx^2*Iyy*psidot*thetadot*cos(theta)*sin(phi)^2*sin(theta)^2 + 2*Ixx*Izz^2*psidot*thetadot*cos(theta)*sin(phi)^2*sin(theta)^2 + 2*Ixx^2*Izz*psidot*thetadot*cos(theta)*sin(phi)^2*sin(theta)^2 + 2*Ixx*Iyy*Izz*psidot*thetadot*cos(theta)^3*sin(phi)^4 - 2*Ixx*Iyy^2*psidot*thetadot*sin(2*theta)*sin(phi)^2*sin(theta) + 2*Ixx^2*Iyy*psidot*thetadot*sin(2*theta)*sin(phi)^2*sin(theta) - 2*Ixx^2*Izz*psidot*thetadot*sin(2*theta)*sin(phi)^2*sin(theta) - 2*Ixx*Izz^2*psidot^2*cos(phi)*cos(theta)^2*sin(phi)^3*sin(theta)^2 - 2*Ixx*Izz^2*psidot^2*cos(phi)^3*cos(theta)^2*sin(phi)*sin(theta)^2 - 2*Ixx*Iyy*Izz*thetadot^2*sin(2*phi)*sin(phi)^2*sin(theta)^2 - 2*Ixx*Iyy*Izz*phidot*thetadot*cos(theta)*sin(theta) - 2*Iyy*Izz*K*l*omega2^2*cos(phi)^2*cos(theta)^2 + 2*Iyy*Izz*K*l*omega4^2*cos(phi)^2*cos(theta)^2 - 2*Ixx*Iyy^2*psidot*thetadot*cos(phi)^2*cos(theta)^3*sin(phi)^2 + 2*Iyy*Izz^2*psidot*thetadot*cos(phi)^2*cos(theta)^3*sin(phi)^2 - 8*Iyy^2*Izz*psidot*thetadot*cos(phi)^2*cos(theta)^3*sin(phi)^2 - 4*Iyy*Izz^2*psidot*thetadot*cos(phi)^2*cos(theta)^3*sin(phi)^4 - 4*Iyy*Izz^2*psidot*thetadot*cos(phi)^4*cos(theta)^3*sin(phi)^2 + 8*Iyy^2*Izz*psidot*thetadot*cos(phi)^2*cos(theta)^3*sin(phi)^4 + 8*Iyy^2*Izz*psidot*thetadot*cos(phi)^4*cos(theta)^3*sin(phi)^2 - 2*Iyy*Izz*K*l*omega2^2*cos(theta)^2*sin(phi)^4 + 2*Iyy*Izz*K*l*omega4^2*cos(theta)^2*sin(phi)^4 - 4*Ixx*Iyy^2*phidot*psidot*cos(phi)*cos(theta)^2*sin(phi)*sin(theta) + 2*Ixx^2*Iyy*phidot*psidot*cos(phi)*cos(theta)^2*sin(phi)*sin(theta) - 2*Ixx^2*Izz*phidot*psidot*cos(phi)*cos(theta)^2*sin(phi)*sin(theta) + 4*Ixx*Iyy*Izz*phidot*thetadot*cos(phi)^2*cos(theta)*sin(theta) + 4*Ixx*Iyy*Izz*phidot*thetadot*cos(theta)*sin(phi)^2*sin(theta) - 2*Iyy*Izz*K*l*omega2^2*cos(phi)^2*cos(theta)^2*sin(phi)^2 + 2*Iyy*Izz*K*l*omega4^2*cos(phi)^2*cos(theta)^2*sin(phi)^2 - 2*Ixx*Iyy*Izz*psidot^2*cos(phi)*cos(theta)^2*sin(phi)*sin(theta)^2 + 2*Ixx*Iyy^2*phidot*psidot*cos(phi)*cos(theta)^2*sin(phi)^3*sin(theta) + 2*Ixx*Iyy^2*phidot*psidot*cos(phi)^3*cos(theta)^2*sin(phi)*sin(theta) + 2*Ixx*Izz^2*phidot*psidot*cos(phi)*cos(theta)^2*sin(phi)^3*sin(theta) + 2*Ixx*Izz^2*phidot*psidot*cos(phi)^3*cos(theta)^2*sin(phi)*sin(theta) + 4*Ixx*Iyy^2*phidot*thetadot*cos(phi)^2*cos(theta)*sin(phi)^2*sin(theta) + 4*Ixx*Izz^2*phidot*thetadot*cos(phi)^2*cos(theta)*sin(phi)^2*sin(theta) - 4*Ixx*Iyy*Izz*psidot*thetadot*cos(theta)*sin(phi)^2*sin(theta)^2 + 2*Ixx*Iyy*Izz*psidot*thetadot*sin(2*theta)*sin(phi)^2*sin(theta) + 2*Ixx*Iyy*Izz*psidot^2*cos(phi)*cos(theta)^2*sin(phi)^3*sin(theta)^2 + 2*Ixx*Iyy*Izz*psidot^2*cos(phi)^3*cos(theta)^2*sin(phi)*sin(theta)^2 + 2*Ixx*Iyy*Izz*psidot*thetadot*cos(phi)^2*cos(theta)^3*sin(phi)^2 - Ixx^2*Iyy*psidot^2*sin(2*theta)*cos(phi)*cos(theta)*sin(phi)*sin(theta) + Ixx^2*Izz*psidot^2*sin(2*theta)*cos(phi)*cos(theta)*sin(phi)*sin(theta) - 4*Ixx*Iyy*Izz*phidot*psidot*cos(phi)*cos(theta)^2*sin(phi)^3*sin(theta) - 4*Ixx*Iyy*Izz*phidot*psidot*cos(phi)^3*cos(theta)^2*sin(phi)*sin(theta) - 8*Ixx*Iyy*Izz*phidot*thetadot*cos(phi)^2*cos(theta)*sin(phi)^2*sin(theta) + 2*Ixx*Iyy*K*l*omega1^2*cos(phi)*cos(theta)*sin(phi)*sin(theta) - 2*Ixx*Iyy*K*l*omega3^2*cos(phi)*cos(theta)*sin(phi)*sin(theta) - 2*Ixx*Izz*K*l*omega1^2*cos(phi)*cos(theta)*sin(phi)*sin(theta) + 2*Ixx*Izz*K*l*omega3^2*cos(phi)*cos(theta)*sin(phi)*sin(theta) - 2*Ixx*Iyy^2*phidot*thetadot*sin(2*phi)*cos(phi)*cos(theta)*sin(phi)*sin(theta) - 2*Ixx*Izz^2*phidot*thetadot*sin(2*phi)*cos(phi)*cos(theta)*sin(phi)*sin(theta) + 4*Ixx*Iyy*Izz*phidot*psidot*cos(phi)*cos(theta)^2*sin(phi)*sin(theta) + 4*Ixx*Iyy*Izz*phidot*thetadot*sin(2*phi)*cos(phi)*cos(theta)*sin(phi)*sin(theta))/(2*Ixx*cos(theta)^2*(- Iyy^2*cos(phi)^2*sin(phi)^2 - Iyy^2*sin(phi)^4 + Iyy^2*sin(phi)^2 + Izz*Iyy*cos(phi)^2*sin(phi)^2 + Izz*Iyy*cos(phi)^2 + Izz*Iyy*sin(phi)^4));
theta_ddot = -(2*Izz^2*psidot^2*cos(phi)^4*cos(theta)^2*sin(theta) + 2*Iyy^2*thetadot^2*cos(phi)^2*sin(phi)^2*sin(theta) + 2*Izz^2*thetadot^2*cos(phi)^2*sin(phi)^2*sin(theta) + 2*Iyy^2*psidot^2*cos(theta)^2*sin(phi)^4*sin(theta) - 2*Izz^2*phidot*psidot*cos(phi)^4*cos(theta)^2 - 2*Iyy^2*phidot*psidot*cos(theta)^2*sin(phi)^4 + 2*Iyy*b*omega1^2*cos(phi)*sin(phi) - 2*Iyy*b*omega2^2*cos(phi)*sin(phi) + 2*Iyy*b*omega3^2*cos(phi)*sin(phi) - 2*Iyy*b*omega4^2*cos(phi)*sin(phi) - 2*Izz*b*omega1^2*cos(phi)*sin(phi) + 2*Izz*b*omega2^2*cos(phi)*sin(phi) - 2*Izz*b*omega3^2*cos(phi)*sin(phi) + 2*Izz*b*omega4^2*cos(phi)*sin(phi) - Ixx*Izz*psidot^2*sin(2*theta)*cos(phi)^2*cos(theta) - 4*Iyy*Izz*thetadot^2*cos(phi)^2*sin(phi)^2*sin(theta) - Ixx*Iyy*psidot^2*sin(2*theta)*cos(theta)*sin(phi)^2 + 2*Izz*K*l*omega1^2*cos(phi)^2*cos(theta) - 2*Izz*K*l*omega3^2*cos(phi)^2*cos(theta) + 2*Izz^2*phidot*thetadot*sin(2*phi)*cos(phi)^2*cos(theta) + 2*Ixx*Izz*phidot*psidot*cos(phi)^2*cos(theta)^2 + 2*Iyy*Izz*phidot*psidot*cos(phi)^4*cos(theta)^2 + 2*Iyy*K*l*omega1^2*cos(theta)*sin(phi)^2 - 2*Iyy*K*l*omega3^2*cos(theta)*sin(phi)^2 - 2*Iyy^2*phidot*thetadot*sin(2*phi)*cos(theta)*sin(phi)^2 + 2*Ixx*Iyy*phidot*psidot*cos(theta)^2*sin(phi)^2 + 2*Iyy*Izz*phidot*psidot*cos(theta)^2*sin(phi)^4 + 2*Iyy^2*psidot^2*cos(phi)^2*cos(theta)^2*sin(phi)^2*sin(theta) + 2*Izz^2*psidot^2*cos(phi)^2*cos(theta)^2*sin(phi)^2*sin(theta) + 2*Iyy^2*phidot*thetadot*cos(phi)*cos(theta)*sin(phi) + 2*Izz^2*phidot*thetadot*cos(phi)*cos(theta)*sin(phi) - 2*Iyy^2*phidot*psidot*cos(phi)^2*cos(theta)^2*sin(phi)^2 - 2*Izz^2*phidot*psidot*cos(phi)^2*cos(theta)^2*sin(phi)^2 - Iyy^2*thetadot^2*sin(2*phi)*cos(phi)*sin(phi)*sin(theta) - Izz^2*thetadot^2*sin(2*phi)*cos(phi)*sin(phi)*sin(theta) - 4*Iyy^2*phidot*thetadot*cos(phi)^3*cos(theta)*sin(phi) - 4*Izz^2*phidot*thetadot*cos(phi)^3*cos(theta)*sin(phi) + 2*Iyy^2*psidot*thetadot*sin(2*theta)*cos(phi)*sin(phi) - 2*Iyy*Izz*phidot*thetadot*sin(2*phi)*cos(phi)^2*cos(theta) + 2*Iyy*Izz*phidot*thetadot*sin(2*phi)*cos(theta)*sin(phi)^2 - 2*Iyy^2*psidot*thetadot*cos(phi)*cos(theta)*sin(phi)*sin(theta) - 2*Izz^2*psidot*thetadot*cos(phi)*cos(theta)*sin(phi)*sin(theta) + 2*Ixx*Iyy*phidot*thetadot*cos(phi)*cos(theta)*sin(phi) - 2*Ixx*Izz*phidot*thetadot*cos(phi)*cos(theta)*sin(phi) - 4*Iyy*Izz*phidot*thetadot*cos(phi)*cos(theta)*sin(phi) + 4*Iyy*Izz*phidot*psidot*cos(phi)^2*cos(theta)^2*sin(phi)^2 + 2*Iyy*Izz*thetadot^2*sin(2*phi)*cos(phi)*sin(phi)*sin(theta) + 8*Iyy*Izz*phidot*thetadot*cos(phi)^3*cos(theta)*sin(phi) - 2*Iyy*K*l*omega2^2*cos(phi)*sin(phi)*sin(theta) + 2*Iyy*K*l*omega4^2*cos(phi)*sin(phi)*sin(theta) + 2*Izz*K*l*omega2^2*cos(phi)*sin(phi)*sin(theta) - 2*Izz*K*l*omega4^2*cos(phi)*sin(phi)*sin(theta) - 2*Ixx*Iyy*psidot*thetadot*sin(2*theta)*cos(phi)*sin(phi) + 2*Ixx*Izz*psidot*thetadot*sin(2*theta)*cos(phi)*sin(phi) - 2*Iyy*Izz*psidot*thetadot*sin(2*theta)*cos(phi)*sin(phi) + 2*Ixx*Iyy*psidot*thetadot*cos(phi)*cos(theta)*sin(phi)*sin(theta) - 2*Ixx*Izz*psidot*thetadot*cos(phi)*cos(theta)*sin(phi)*sin(theta) + 4*Iyy*Izz*psidot*thetadot*cos(phi)*cos(theta)*sin(phi)*sin(theta))/(2*cos(theta)*(- Iyy^2*cos(phi)^2*sin(phi)^2 - Iyy^2*sin(phi)^4 + Iyy^2*sin(phi)^2 + Izz*Iyy*cos(phi)^2*sin(phi)^2 + Izz*Iyy*cos(phi)^2 + Izz*Iyy*sin(phi)^4));
psi_ddot = (2*Iyy*b*omega1^2 - 2*Iyy*b*omega2^2 + 2*Iyy*b*omega3^2 - 2*Iyy*b*omega4^2 - Iyy^2*thetadot^2*sin(2*phi)*sin(theta) - 2*Iyy*b*omega1^2*sin(phi)^2 + 2*Iyy*b*omega2^2*sin(phi)^2 - 2*Iyy*b*omega3^2*sin(phi)^2 + 2*Iyy*b*omega4^2*sin(phi)^2 + 2*Izz*b*omega1^2*sin(phi)^2 - 2*Izz*b*omega2^2*sin(phi)^2 + 2*Izz*b*omega3^2*sin(phi)^2 - 2*Izz*b*omega4^2*sin(phi)^2 + 2*Iyy^2*psidot*thetadot*sin(2*theta) + 2*Iyy^2*phidot*thetadot*cos(theta) - 2*Iyy^2*phidot*thetadot*cos(theta)*sin(phi)^2 - 2*Izz^2*phidot*thetadot*cos(theta)*sin(phi)^2 - 2*Iyy*K*l*omega2^2*sin(theta) + 2*Iyy*K*l*omega4^2*sin(theta) - 2*Ixx*Iyy*psidot*thetadot*sin(2*theta) + Iyy^2*thetadot^2*sin(2*phi)*sin(phi)^2*sin(theta) + Izz^2*thetadot^2*sin(2*phi)*sin(phi)^2*sin(theta) - 2*Iyy^2*psidot*thetadot*sin(2*theta)*sin(phi)^2 + 2*Iyy^2*thetadot^2*cos(phi)*sin(phi)*sin(theta) - 2*Iyy^2*psidot*thetadot*cos(theta)*sin(theta) + 2*Ixx*Iyy*phidot*thetadot*cos(theta) - 2*Iyy*Izz*phidot*thetadot*cos(theta) - 2*Iyy^2*thetadot^2*cos(phi)*sin(phi)^3*sin(theta) - 2*Izz^2*thetadot^2*cos(phi)*sin(phi)^3*sin(theta) + Iyy*Izz*thetadot^2*sin(2*phi)*sin(theta) - 4*Iyy^2*phidot*thetadot*cos(phi)^2*cos(theta) - 2*Izz^2*psidot^2*cos(phi)*cos(theta)^2*sin(phi)^3*sin(theta) - 2*Izz^2*psidot^2*cos(phi)^3*cos(theta)^2*sin(phi)*sin(theta) - 2*Iyy*Izz*thetadot^2*sin(2*phi)*sin(phi)^2*sin(theta) + 2*Iyy^2*phidot*psidot*cos(phi)*cos(theta)^2*sin(phi)^3 + 2*Iyy^2*phidot*psidot*cos(phi)^3*cos(theta)^2*sin(phi) + 2*Izz^2*phidot*psidot*cos(phi)*cos(theta)^2*sin(phi)^3 + 2*Izz^2*phidot*psidot*cos(phi)^3*cos(theta)^2*sin(phi) + 4*Iyy^2*phidot*thetadot*cos(phi)^2*cos(theta)*sin(phi)^2 + 4*Izz^2*phidot*thetadot*cos(phi)^2*cos(theta)*sin(phi)^2 + 2*Iyy*K*l*omega2^2*sin(phi)^2*sin(theta) - 2*Iyy*K*l*omega4^2*sin(phi)^2*sin(theta) - 2*Izz*K*l*omega2^2*sin(phi)^2*sin(theta) + 2*Izz*K*l*omega4^2*sin(phi)^2*sin(theta) + 2*Ixx*Iyy*psidot*thetadot*sin(2*theta)*sin(phi)^2 - 2*Ixx*Izz*psidot*thetadot*sin(2*theta)*sin(phi)^2 + 2*Iyy*Izz*psidot*thetadot*sin(2*theta)*sin(phi)^2 - 2*Iyy*Izz*thetadot^2*cos(phi)*sin(phi)*sin(theta) + 2*Ixx*Iyy*psidot*thetadot*cos(theta)*sin(theta) + 2*Iyy*Izz*psidot*thetadot*cos(theta)*sin(theta) + 2*Iyy^2*psidot^2*cos(phi)*cos(theta)^2*sin(phi)*sin(theta) + 4*Iyy*Izz*thetadot^2*cos(phi)*sin(phi)^3*sin(theta) - 4*Iyy^2*phidot*psidot*cos(phi)*cos(theta)^2*sin(phi) + 4*Iyy*Izz*phidot*thetadot*cos(phi)^2*cos(theta) + 2*Iyy^2*psidot*thetadot*cos(theta)*sin(phi)^2*sin(theta) + 2*Izz^2*psidot*thetadot*cos(theta)*sin(phi)^2*sin(theta) - 2*Ixx*Iyy*phidot*thetadot*cos(theta)*sin(phi)^2 + 2*Ixx*Izz*phidot*thetadot*cos(theta)*sin(phi)^2 + 4*Iyy*Izz*phidot*thetadot*cos(theta)*sin(phi)^2 - 4*Iyy*Izz*phidot*psidot*cos(phi)*cos(theta)^2*sin(phi)^3 - 4*Iyy*Izz*phidot*psidot*cos(phi)^3*cos(theta)^2*sin(phi) - 8*Iyy*Izz*phidot*thetadot*cos(phi)^2*cos(theta)*sin(phi)^2 - Ixx*Iyy*psidot^2*sin(2*theta)*cos(phi)*cos(theta)*sin(phi) + Ixx*Izz*psidot^2*sin(2*theta)*cos(phi)*cos(theta)*sin(phi) - 2*Iyy*Izz*psidot^2*cos(phi)*cos(theta)^2*sin(phi)*sin(theta) + 2*Iyy*K*l*omega1^2*cos(phi)*cos(theta)*sin(phi) - 2*Iyy*K*l*omega3^2*cos(phi)*cos(theta)*sin(phi) - 2*Izz*K*l*omega1^2*cos(phi)*cos(theta)*sin(phi) + 2*Izz*K*l*omega3^2*cos(phi)*cos(theta)*sin(phi) - 2*Iyy^2*phidot*thetadot*sin(2*phi)*cos(phi)*cos(theta)*sin(phi) - 2*Izz^2*phidot*thetadot*sin(2*phi)*cos(phi)*cos(theta)*sin(phi) + 2*Ixx*Iyy*phidot*psidot*cos(phi)*cos(theta)^2*sin(phi) - 2*Ixx*Izz*phidot*psidot*cos(phi)*cos(theta)^2*sin(phi) + 4*Iyy*Izz*phidot*psidot*cos(phi)*cos(theta)^2*sin(phi) - 2*Ixx*Iyy*psidot*thetadot*cos(theta)*sin(phi)^2*sin(theta) + 2*Ixx*Izz*psidot*thetadot*cos(theta)*sin(phi)^2*sin(theta) - 4*Iyy*Izz*psidot*thetadot*cos(theta)*sin(phi)^2*sin(theta) + 2*Iyy*Izz*psidot^2*cos(phi)*cos(theta)^2*sin(phi)^3*sin(theta) + 2*Iyy*Izz*psidot^2*cos(phi)^3*cos(theta)^2*sin(phi)*sin(theta) + 4*Iyy*Izz*phidot*thetadot*sin(2*phi)*cos(phi)*cos(theta)*sin(phi))/(2*cos(theta)^2*(- Iyy^2*cos(phi)^2*sin(phi)^2 - Iyy^2*sin(phi)^4 + Iyy^2*sin(phi)^2 + Izz*Iyy*cos(phi)^2*sin(phi)^2 + Izz*Iyy*cos(phi)^2 + Izz*Iyy*sin(phi)^4));

if ((z_ddot<0 && z ==0) || z<0)
    rest=1;
    z_ddot=0;    
end

end

== matlab function cable_driven_parallel_robot2022/Actuators-CableTension-MovingPlatform/QuadRotor3/Subsystem/Subsystem/MATLAB Function ==
  data: rest0 input; rest output; init0 input; init output
function [rest,init] = fcn(rest0,init0)

if rest0==1
    rest=rest0;
    init=0;
else
  rest = rest0;
  init = init0;

end

== matlab function cable_driven_parallel_robot2022/Actuators-CableTension-MovingPlatform/QuadRotor3/Subsystem/Subsystem1/MATLAB Function ==
  data: rest0 input; rest output; init0 input; init output
function [rest,init] = fcn(rest0,init0)

if rest0==1
    rest=rest0;
    init=0;
else
  rest = rest0;
  init = init0;

end

== matlab function cable_driven_parallel_robot2022/Actuators-CableTension-MovingPlatform/MATLAB Function ==
  data: QR_Vel_U1 input; Vmin output; QR_Vel_U2 input; QR_Vel_U3 input; QR_Vel_U4 input; MP_Vel input; MR_Vel_L1 input; MR_Vel_L2 input; MR_Vel_L3 input; MR_Vel_L4 input; isTension input
function Vmin   = fcn(QR_Vel_U1,QR_Vel_U2,QR_Vel_U3,QR_Vel_U4,MP_Vel,MR_Vel_L1,MR_Vel_L2,MR_Vel_L3,MR_Vel_L4,isTension)
Vmin=zeros(3,1);
Vx= [QR_Vel_U1(1),QR_Vel_U2(1),QR_Vel_U3(1),QR_Vel_U4(1),MP_Vel(1),MR_Vel_L1(1),MR_Vel_L2(1),MR_Vel_L3(1),MR_Vel_L4(1)];
Vx_abs=abs(Vx);
Vx_max=max(Vx_abs);


Vx_abs=[abs(QR_Vel_U1(1)) + not(isTension(1))*Vx_max, ...
        abs(QR_Vel_U2(1)) + not(isTension(2))*Vx_max, ...
        abs(QR_Vel_U3(1)) + not(isTension(3))*Vx_max, ...
        abs(QR_Vel_U4(1)) + not(isTension(4))*Vx_max, ...
        abs(MP_Vel(1))    + not(or(sum(isTension),0))*Vx_max, ...
        abs(MR_Vel_L1(1)) + not(isTension(5))*Vx_max, ...
        abs(MR_Vel_L2(1)) + not(isTension(6))*Vx_max, ...
        abs(MR_Vel_L3(1)) + not(isTension(7))*Vx_max, ...
        abs(MR_Vel_L4(1)) + not(isTension(8))*Vx_max];
    
 [~, X_idx]=min(Vx_abs);
 
 %%%%%%%%%%%%%%%%%%%%%%%%%%%%%%%%%%%%%%%%%%%%%%%%%%%%%%%%%%%%%%%%%%%%%%%%%
 
Vy= [QR_Vel_U1(2),QR_Vel_U2(2),QR_Vel_U3(2),QR_Vel_U4(2),MP_Vel(2),MR_Vel_L1(2),MR_Vel_L2(2),MR_Vel_L3(2),MR_Vel_L4(2)];
Vy_abs=abs(Vy);
Vy_max=max(Vy_abs);


Vy_abs=[abs(QR_Vel_U1(2)) + not(isTension(1))*Vy_max, ...
        abs(QR_Vel_U2(2)) + not(isTension(2))*Vy_max, ...
        abs(QR_Vel_U3(2)) + not(isTension(3))*Vy_max, ...
        abs(QR_Vel_U4(2)) + not(isTension(4))*Vy_max, ...
        abs(MP_Vel(2))    + not(or(sum(isTension),0))*Vy_max, ...
        abs(MR_Vel_L1(2)) + not(isTension(5))*Vy_max, ...
        abs(MR_Vel_L2(2)) + not(isTension(6))*Vy_max, ...
        abs(MR_Vel_L3(2)) + not(isTension(7))*Vy_max, ...
        abs(MR_Vel_L4(2)) + not(isTension(8))*Vy_max];
    
 [~, Y_idx]=min(Vy_abs);
 
%%%%%%%%%%%%%%%%%%%%%%%%%%%%%%%%%%%%%%%%%%%%%%%%%%%%%%%%%%%%%%%%%%%%%%%%%%
Vz= [QR_Vel_U1(3),QR_Vel_U2(3),QR_Vel_U3(3),QR_Vel_U4(3),MP_Vel(3),MR_Vel_L1(3),MR_Vel_L2(3),MR_Vel_L3(3),MR_Vel_L4(3)];
Vz_abs=abs(Vz);
Vz_max=max(Vz_abs);


Vz_abs=[abs(QR_Vel_U1(2)) + not(isTension(1))*Vz_max, ...
        abs(QR_Vel_U2(2)) + not(isTension(2))*Vz_max, ...
        abs(QR_Vel_U3(2)) + not(isTension(3))*Vz_max, ...
        abs(QR_Vel_U4(2)) + not(isTension(4))*Vz_max, ...
        abs(MP_Vel(2))    + not(or(sum(isTension),0))*Vz_max, ...
        abs(MR_Vel_L1(2)) + not(isTension(5))*Vz_max, ...
        abs(MR_Vel_L2(2)) + not(isTension(6))*Vz_max, ...
        abs(MR_Vel_L3(2)) + not(isTension(7))*Vz_max, ...
        abs(MR_Vel_L4(2)) + not(isTension(8))*Vz_max];
    
 [~, Z_idx]=min(Vz_abs);
 
 Vmin(1) = Vx(X_idx);
 Vmin(2) = Vy(Y_idx);
 Vmin(3) = Vz(Z_idx);

== matlab function cable_driven_parallel_robot2022/Actuators-CableTension-MovingPlatform/Moving Platform/Moving Platform/MATLAB Function3 ==
  settings: updateMethod=DISCRETE
  data: angle input; delta output
function delta = fcn(angle)

persistent angle_previous

if isempty(angle_previous)
  angle_previous = 0;
  delta = atan2(sin(angle-angle_previous),cos(angle-angle_previous));
  angle_previous=angle;
  return
end

  delta = atan2(sin(angle-angle_previous),cos(angle-angle_previous));
  angle_previous = angle;

== matlab function cable_driven_parallel_robot2022/Actuators-CableTension-MovingPlatform/Moving Platform/Moving Platform/MATLAB Function4 ==
  settings: updateMethod=DISCRETE
  data: angle input; delta output
function delta = fcn(angle)

persistent angle_previous

if isempty(angle_previous)
  angle_previous = 0;
  delta = atan2(sin(angle-angle_previous),cos(angle-angle_previous));
  angle_previous=angle;
  return
end

  delta = atan2(sin(angle-angle_previous),cos(angle-angle_previous));
  angle_previous = angle;

== matlab function cable_driven_parallel_robot2022/Actuators-CableTension-MovingPlatform/Moving Platform/Moving Platform/MATLAB Function5 ==
  settings: updateMethod=DISCRETE
  data: angle input; delta output
function delta = fcn(angle)

persistent angle_previous

if isempty(angle_previous)
  angle_previous = 0;
  delta = atan2(sin(angle-angle_previous),cos(angle-angle_previous));
  angle_previous=angle;
  return
end

  delta = atan2(sin(angle-angle_previous),cos(angle-angle_previous));
  angle_previous = angle;

== matlab function cable_driven_parallel_robot2022/Actuators-CableTension-MovingPlatform/2 Wheels Diffrential Mobile Robot/2 Wheels Diffrential Mobile Robot/2 Wheels Diffrential Mobile Robot ==
  settings: updateMethod=DISCRETE
  data: TR input; TL input; Tx input; Ty input; Tz input; Jr input; mr input; r input; ax output; ay output; az output; alpha_r output; WT input
function [ax,ay,az,alpha_r] = fcn(TR,TL,Tx,Ty,Tz,Jr,mr,r,WT)

g=9.81;

ax = ((TR/r)+(TL/r)+Tx)/mr;
ay = (Ty)/mr;
az = (Tz -mr*g)/mr;

alpha_r = ((TR-TL)*(WT/2*r))/Jr;
